simulink model "ecu_sensors"  (R2026a)
settings: Solver=FixedStepDiscrete  StopTime=10  FixedStep=0.001  SampleTimeConstraint=STIndependent
Description:
  | Sensor conversion and range faults. Source of truth for firmware/gen/ecu_sensors.
settings Model: Creator=jj1001000  LastModifiedBy=jj1001000
settings OptimizationCC: DefaultUnderspecifiedDataType=single
settings DebuggingCC: ParameterPrecisionLossMsg=none
settings HardwareCC: ProdLargestAtomicInteger=Long  ProdLargestAtomicFloat=Double  ProdHWDeviceType=ARM Compatible->ARM Cortex-M
settings RTWCC: SystemTargetFile=ert.tlc  GenCodeOnly=on  Description=Embedded Coder
settings ERTTargetCC: UtilityFuncGeneration=Shared location  IncludeMdlTerminateFcn=off  CodeInterfacePackaging=Reusable function  SupportNonFinite=off

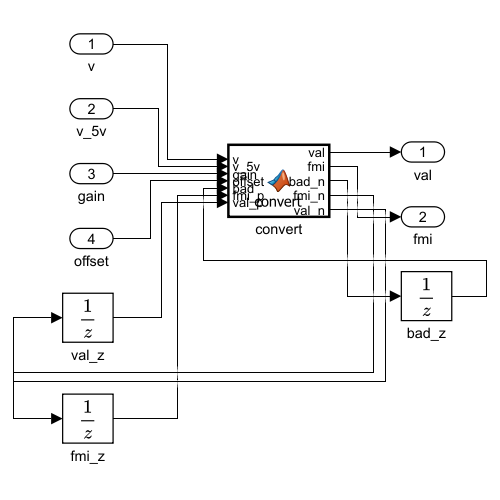
[thumbnail: Simulink's stored preview of the top-level diagram]
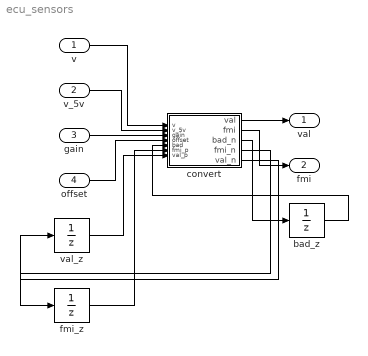
== system ecu_sensors ==
  v : Inport  OutDataTypeStr=single  PortDimensions=5
  v_5v : Inport  Port=2  OutDataTypeStr=single  PortDimensions=1
  gain : Inport  Port=3  OutDataTypeStr=single  PortDimensions=6
  offset : Inport  Port=4  OutDataTypeStr=single  PortDimensions=6
  bad_z : UnitDelay  InitialCondition=zeros(5,1)  SampleTime=-1
  convert : MATLAB Function  TreatAsAtomicUnit=on
  fmi_z : UnitDelay  InitialCondition=zeros(5,1)  SampleTime=-1
  val_z : UnitDelay  InitialCondition=[90;300;1000;100;0]  SampleTime=-1
  val : Outport  OutDataTypeStr=single
  fmi : Outport  Port=2  OutDataTypeStr=uint8
  wires:
  v/1 -> convert/1(v)
  v_5v/1 -> convert/2(v_5v)
  gain/1 -> convert/3(gain)
  offset/1 -> convert/4(offset)
  val_z/1 -> convert/7(val_p)
  fmi_z/1 -> convert/6(fmi_p)
  convert/1(val) -> val/1
  convert/2(fmi) -> fmi/1
  convert/3(bad_n) -> bad_z/1
  convert/4(fmi_n) -> fmi_z/1
  convert/5(val_n) -> val_z/1
  bad_z/1 -> convert/5(bad)

== matlab function ecu_sensors/convert ==
  data: v input single; val output single; v_5v input single; gain input single; offset input single; bad input uint16; fmi_p input uint8; val_p input single; fmi output uint8; bad_n output uint16; fmi_n output uint8; val_n output single
function [val, fmi, bad_n, fmi_n, val_n] = convert(v, v_5v, gain, offset, bad, fmi_p, val_p)
%#codegen
DEF = single([90 300 1000 100 0]); VLO = single([0.100000001 0.200000003 0.200000003 0.200000003 0.200000003]); SLO = single([0 0 0 50 0]); SHI = single([0 1000 1800 400 100]);
NT = single([-40 -30 -20 -10 0 10 20 30 40 50 60 70 80 90 100 110 120 130 140 150]); NR = single([45313 26114 15462 9397 5896 3792 2500 1707 1175 834 596 436 323 243 187 144 113 89 71 57]);
v5 = v_5v * gain(6) + offset(6);
if ~(v5 >= single(4.5) && v5 <= single(5.5))   % supply fault: use nominal
    v5 = single(5);
end
bad_n = bad; fmi_n = fmi_p; val_n = val_p;
for i = 1:5
    vr = (v(i) * gain(i) + offset(i)) * single(5) / v5;
    if ~(vr <= single(4.80000019))                     % NaN reads high
        now = uint8(3);
    elseif vr < VLO(i)
        now = uint8(4);
    else
        now = uint8(0);
    end
    % the count is time spent disagreeing with the latched state
    if (now ~= 0) ~= (fmi_n(i) ~= 0)
        bad_n(i) = bad_n(i) + uint16(1);
        if bad_n(i) >= uint16(100)
            fmi_n(i) = now;
            bad_n(i) = uint16(0);
        end
    else
        bad_n(i) = uint16(0);
        if now ~= 0
            fmi_n(i) = now;
        end
    end
    % faulted: the default; out of range but not yet latched: hold
    if fmi_n(i) ~= 0
        val_n(i) = DEF(i);
    elseif now == 0
        if i == 1                              % coolant NTC, Bosch table in ln(R)
            r = single(2490) * vr / (single(5) - vr);
            if r < single(260000)
                r = r * single(260000) / (single(260000) - r);
            else
                r = single(1e9);
            end
            if ~(r < NR(1))
                val_n(i) = NT(1);
            elseif r <= NR(20)
                val_n(i) = NT(20);
            else
                k = int32(1);
                while r <= NR(k + 1)
                    k = k + int32(1);
                end
                val_n(i) = NT(k) + (NT(k + 1) - NT(k)) * (log(NR(k) / r) / log(NR(k) / NR(k + 1)));
            end
        else
            val_n(i) = SLO(i) + (vr - single(0.5)) / single(4) * (SHI(i) - SLO(i));
        end
    end
end
val = val_n; fmi = fmi_n;
